simulink model "CartDataReader"  (R2026b)
settings: Solver=VariableStepAuto
libraries: raspberrypiCommlib x1
settings Model: Creator=alex  LastModifiedBy=super

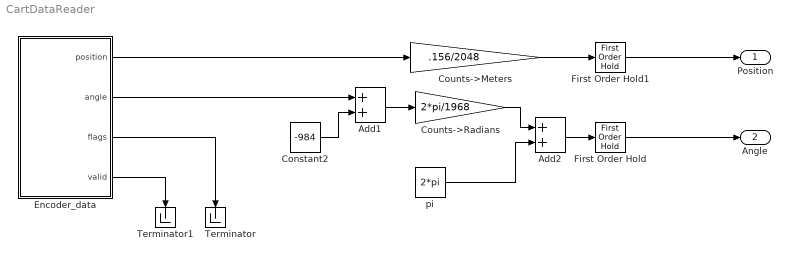
== system CartDataReader ==
  Add1 : Sum
  Add2 : Sum
  Constant2 : Constant  Value=-984
  Counts->Meters : Gain  Gain=.156/2048  SaturateOnIntegerOverflow=on  OutDataTypeStr=Inherit: Same as input  ParamDataTypeStr=Inherit: Same as input
  Counts->Radians : Gain  Gain=2*pi/1968  SaturateOnIntegerOverflow=on  OutDataTypeStr=Inherit: Same as input  ParamDataTypeStr=Inherit: Same as input
  Encoder_data : Subsystem
  First Order Hold : FirstOrderHold  InitialOutput=pi  OutputAlgorithm=Fast (Minimize Error)  ErrorTolerance=inf
  First Order Hold1 : FirstOrderHold  OutputAlgorithm=Fast (Minimize Error)  ErrorTolerance=inf
  Terminator : Terminator
  Terminator1 : Terminator
  pi : Constant  Value=2*pi
  Position : Outport
  Angle : Outport  Port=2
  wires:
  pi/1 -> Add2/2
  Counts->Radians/1 -> Add2/1
  Counts->Meters/1 -> First Order Hold1/1
  Encoder_data/2(angle) -> Add1/1
  Encoder_data/1(position) -> Counts->Meters/1
  Add1/1 -> Counts->Radians/1
  Constant2/1 -> Add1/2
  Encoder_data/4(valid) -> Terminator1/1
  Encoder_data/3(flags) -> Terminator/1
  Add2/1 -> First Order Hold/1
  First Order Hold/1 -> Angle/1
  First Order Hold1/1 -> Position/1

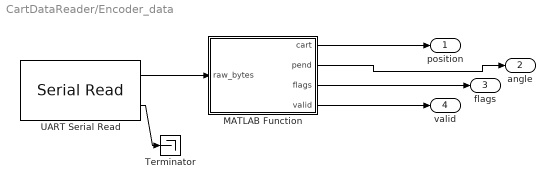
== system CartDataReader/Encoder_data ==
  MATLAB Function : MATLAB Function  TreatAsAtomicUnit=on
  Terminator : Terminator
  UART Serial Read : raspberrypiCommlib/Serial Read  board=Pi 5 Model  SCIModule_=/dev/ttyAMA0  Baudrate_=230400  Parity=None  StopBits_=1  HardwareFlowControl=None  ByteOrder=LittleEndian  DataLength=12  DataType=uint8  OutputStatus=on  SampleTime=0.001  blockPlatform=RaspberryPi
  position : Outport
  angle : Outport  Port=2
  flags : Outport  Port=3
  valid : Outport  Port=4
  wires:
  UART Serial Read/1 -> MATLAB Function/1(raw_bytes)
  MATLAB Function/1(cart) -> position/1
  MATLAB Function/4(valid) -> valid/1
  MATLAB Function/2(pend) -> angle/1
  MATLAB Function/3(flags) -> flags/1
  UART Serial Read/2 -> Terminator/1

== matlab function CartDataReader/Encoder_data/MATLAB Function ==
  data: raw_bytes input; cart output; pend output; flags output; valid output
function [cart, pend, flags, valid] = decode_packet(raw_bytes)
% 12-byte measurement from the ESP32: A5 5A, cart int32 LE, pend int32 LE, flags, XOR(bytes 3..11).
% A missing, short or misaligned read (valid = false) keeps the last good values, so a lost
% byte never feeds garbage counts to the controller.
persistent last_cart last_pend last_flags
if isempty(last_cart)
    last_cart = 0; last_pend = 0; last_flags = 0;
end
b = uint8(raw_bytes(1:12));
header_ok = (b(1) == 165) && (b(2) == 90);
xor_val = uint8(0);
for i = 3:11
    xor_val = bitxor(xor_val, b(i));
end
valid = boolean(header_ok && (xor_val == b(12)));
if valid
    cart_i32 = typecast(b(3:6), 'int32');
    pend_i32 = typecast(b(7:10), 'int32');
    last_cart  = double(cart_i32(1));
    last_pend  = double(pend_i32(1));
    last_flags = double(b(11));
end
cart  = last_cart;
pend  = last_pend;
flags = last_flags;
end
